simulink model "nms_sim_2D_cost"  (R2024b)
settings: Solver=ode15s  StartTime=0.0  StopTime=t_sim  MaxStep=dt_max  EnableMultiTasking=on
values from neighbouring files (symbols this model uses):
  a_BFSH = param_ctrl(35)*1    [setCtrlPar_optim_CPGreflex2001_2D.m]
  a_GAS = param_ctrl(37)*1    [setCtrlPar_optim_CPGreflex2001_2D.m]
  a_GLU = param_ctrl(31)*1    [setCtrlPar_optim_CPGreflex2001_2D.m]
  a_HAM = param_ctrl(33)*1    [setCtrlPar_optim_CPGreflex2001_2D.m]
  a_HFL = param_ctrl(32)*1    [setCtrlPar_optim_CPGreflex2001_2D.m]
  a_RF = param_ctrl(34)*1    [setCtrlPar_optim_CPGreflex2001_2D.m]
  a_SOL = param_ctrl(38)*1    [setCtrlPar_optim_CPGreflex2001_2D.m]
  a_TA = param_ctrl(39)*1    [setCtrlPar_optim_CPGreflex2001_2D.m]
  a_VAS = param_ctrl(36)*1    [setCtrlPar_optim_CPGreflex2001_2D.m]
  ai = param_ctrl(96)*2.0    [setCtrlPar_optim_CPGreflex2001_2D.m]
  b_BFSH = param_ctrl(52)*.51    [setCtrlPar_optim_CPGreflex2001_2D.m]
  b_BFSHGAS = param_ctrl(55)*.51    [setCtrlPar_optim_CPGreflex2001_2D.m]
  b_BFSHHAM = param_ctrl(54)*.51    [setCtrlPar_optim_CPGreflex2001_2D.m]
  b_BFSHVAS = param_ctrl(53)*.51    [setCtrlPar_optim_CPGreflex2001_2D.m]
  b_GAS = param_ctrl(59)*.51    [setCtrlPar_optim_CPGreflex2001_2D.m]
  b_GASBFSH = param_ctrl(60)*.51    [setCtrlPar_optim_CPGreflex2001_2D.m]
  b_GASSOL = param_ctrl(61)*.51    [setCtrlPar_optim_CPGreflex2001_2D.m]
  b_GLU = param_ctrl(40)*.51    [setCtrlPar_optim_CPGreflex2001_2D.m]
  b_GLUHAM = param_ctrl(42)*.51    [setCtrlPar_optim_CPGreflex2001_2D.m]
  b_GLUHFL = param_ctrl(41)*.51    [setCtrlPar_optim_CPGreflex2001_2D.m]
  b_HAM = param_ctrl(46)*.51    [setCtrlPar_optim_CPGreflex2001_2D.m]
  b_HAMBFSH = param_ctrl(48)*.51    [setCtrlPar_optim_CPGreflex2001_2D.m]
  b_HAMGLU = param_ctrl(47)*.51    [setCtrlPar_optim_CPGreflex2001_2D.m]
  b_HFL = param_ctrl(43)*.51    [setCtrlPar_optim_CPGreflex2001_2D.m]
  b_HFLGLU = param_ctrl(44)*.51    [setCtrlPar_optim_CPGreflex2001_2D.m]
  b_HFLRF = param_ctrl(45)*.51    [setCtrlPar_optim_CPGreflex2001_2D.m]
  b_RF = param_ctrl(49)*.51    [setCtrlPar_optim_CPGreflex2001_2D.m]
  b_RFHFL = param_ctrl(50)*.51    [setCtrlPar_optim_CPGreflex2001_2D.m]
  b_RFVAS = param_ctrl(51)*.51    [setCtrlPar_optim_CPGreflex2001_2D.m]
  b_SOL = param_ctrl(62)*.51    [setCtrlPar_optim_CPGreflex2001_2D.m]
  b_SOLGAS = param_ctrl(64)*.51    [setCtrlPar_optim_CPGreflex2001_2D.m]
  b_SOLTA = param_ctrl(63)*.51    [setCtrlPar_optim_CPGreflex2001_2D.m]
  b_TA = param_ctrl(65)*.51    [setCtrlPar_optim_CPGreflex2001_2D.m]
  b_TASOL = param_ctrl(66)*.51    [setCtrlPar_optim_CPGreflex2001_2D.m]
  b_VAS = param_ctrl(56)*.51    [setCtrlPar_optim_CPGreflex2001_2D.m]
  b_VASBFSH = param_ctrl(57)*.51    [setCtrlPar_optim_CPGreflex2001_2D.m]
  b_VASRF = param_ctrl(58)*.51    [setCtrlPar_optim_CPGreflex2001_2D.m]
  bias = param_ctrl(97)*2.5    [setCtrlPar_optim_CPGreflex2001_2D.m]
  c = 0.05    [nms_MS_2D_scaled.m]
  c_jointstop = 0.3 / (pi/180)    (= 17.1887338539)    [nms_MS_2D_scaled.m]
  D12_F = 0.16    *scaleL_JPhys    [nms_MechInit_2D_scaleSkel.m]
  D12_S = 0.2460	*sub_height    [nms_MechInit_2D_scaleSkel.m]
  D12_T = 0.2450  *sub_height    [nms_MechInit_2D_scaleSkel.m]
  D12y_F = 0.039  *sub_height    [nms_MechInit_2D_scaleSkel.m]
  D12z_HAT = 0.1    [nms_MS_2D_scaled.m]
  D13_F = 0.20    *scaleL_JPhys    [nms_MechInit_2D_scaleSkel.m]
  D1G_F = 0.14    *scaleL_JPhys    [nms_MechInit_2D_scaleSkel.m]
  D1G_HAT = 0.35  *scaleL_JPhys    [nms_MechInit_2D_scaleSkel.m]
  D1G_S = (0.3 - D12y_F/4)	*scaleL_JPhys    [nms_MechInit_2D_scaleSkel.m]
  D1G_T = (0.3 - D12y_F/4)	*scaleL_JPhys    [nms_MechInit_2D_scaleSkel.m]
  D1Gy_F = D12y_F*D1G_F/D12_F    (= 0.07)    [nms_MechInit_2D_scaleSkel.m]
  d_BFSH = param_ctrl(26)*1    [setCtrlPar_optim_CPGreflex2001_2D.m]
  d_GAS = param_ctrl(28)*1    [setCtrlPar_optim_CPGreflex2001_2D.m]
  d_GLU = param_ctrl(22)*1    [setCtrlPar_optim_CPGreflex2001_2D.m]
  d_HAM = param_ctrl(24)*1    [setCtrlPar_optim_CPGreflex2001_2D.m]
  d_HFL = param_ctrl(23)*1    [setCtrlPar_optim_CPGreflex2001_2D.m]
  d_RF = param_ctrl(25)*1    [setCtrlPar_optim_CPGreflex2001_2D.m]
  d_SOL = param_ctrl(29)*1    [setCtrlPar_optim_CPGreflex2001_2D.m]
  d_TA = param_ctrl(30)*1    [setCtrlPar_optim_CPGreflex2001_2D.m]
  d_VAS = param_ctrl(27)*1    [setCtrlPar_optim_CPGreflex2001_2D.m]
  DeltaThRef = 5e-3    (= 0.005)    [nms_MS_2D_scaled.m]
  dloptBFSH = 3.0    (= 3)    [setCtrlPar_optim_CPGreflex2001_2D.m]
  dloptGAS = 3.0    (= 3)    [setCtrlPar_optim_CPGreflex2001_2D.m]
  dloptGLU = 3.0    (= 3)    [setCtrlPar_optim_CPGreflex2001_2D.m]
  dloptHAM = 3.0    (= 3)    [setCtrlPar_optim_CPGreflex2001_2D.m]
  dloptHFL = 3.0    (= 3)    [setCtrlPar_optim_CPGreflex2001_2D.m]
  dloptRF = 3.0    (= 3)    [setCtrlPar_optim_CPGreflex2001_2D.m]
  dloptSOL = 3.0    (= 3)    [setCtrlPar_optim_CPGreflex2001_2D.m]
  dloptTA = 3.0    (= 3)    [setCtrlPar_optim_CPGreflex2001_2D.m]
  dloptVAS = 3.0    (= 3)    [setCtrlPar_optim_CPGreflex2001_2D.m]
  ec_BFSH = param_ctrl(80)*0.15    [setCtrlPar_optim_CPGreflex2001_2D.m]
  ec_GAS = param_ctrl(82)*0.15    [setCtrlPar_optim_CPGreflex2001_2D.m]
  ec_GLU = param_ctrl(76)*0.15    [setCtrlPar_optim_CPGreflex2001_2D.m]
  ec_HAM = param_ctrl(78)*0.15    [setCtrlPar_optim_CPGreflex2001_2D.m]
  ec_HFL = param_ctrl(77)*0.15    [setCtrlPar_optim_CPGreflex2001_2D.m]
  ec_RF = param_ctrl(79)*0.15    [setCtrlPar_optim_CPGreflex2001_2D.m]
  ec_TA = param_ctrl(84)*0.15    [setCtrlPar_optim_CPGreflex2001_2D.m]
  ec_VAS = param_ctrl(81)*0.15    [setCtrlPar_optim_CPGreflex2001_2D.m]
  eref = 0.04    [nms_MS_2D_scaled.m]
  eref_GAS = 0.1    [nms_MS_2D_scaled.m]
  eref_SOL = 0.1    [nms_MS_2D_scaled.m]
  es_BFSH = param_ctrl(89)*0.15    [setCtrlPar_optim_CPGreflex2001_2D.m]
  es_GAS = param_ctrl(91)*0.15    [setCtrlPar_optim_CPGreflex2001_2D.m]
  es_GLU = param_ctrl(85)*0.15    [setCtrlPar_optim_CPGreflex2001_2D.m]
  es_HAM = param_ctrl(87)*0.15    [setCtrlPar_optim_CPGreflex2001_2D.m]
  es_HFL = param_ctrl(86)*0.15    [setCtrlPar_optim_CPGreflex2001_2D.m]
  es_RF = param_ctrl(88)*0.15    [setCtrlPar_optim_CPGreflex2001_2D.m]
  es_TA = param_ctrl(93)*0.15    [setCtrlPar_optim_CPGreflex2001_2D.m]
  es_VAS = param_ctrl(90)*0.15    [setCtrlPar_optim_CPGreflex2001_2D.m]
  FmaxBFSH = 350    [nms_MS_2D_scaled.m]
  FmaxGAS = 2000    [nms_MS_2D_scaled.m]
  FmaxGLU = 4000    [nms_MS_2D_scaled.m]
  FmaxHAM = 2000    [nms_MS_2D_scaled.m]
  FmaxHFL = 2000    [nms_MS_2D_scaled.m]
  FmaxRF = 850    [nms_MS_2D_scaled.m]
  FmaxSOL = 4000    [nms_MS_2D_scaled.m]
  FmaxTA = 800    [nms_MS_2D_scaled.m]
  FmaxVAS = 5000    [nms_MS_2D_scaled.m]
  g = 9.81    [nms_MS_2D_scaled.m]
  gamma_4 = param_ctrl(11) * 1.7    [setCtrlPar_optim_CPGreflexsynergy2023_2D.m]
  h_BFSH = param_ctrl(71)*.1    [setCtrlPar_optim_CPGreflex2001_2D.m]
  h_GAS = param_ctrl(73)*.1    [setCtrlPar_optim_CPGreflex2001_2D.m]
  h_GLU = param_ctrl(67)*.1    [setCtrlPar_optim_CPGreflex2001_2D.m]
  h_HAM = param_ctrl(69)*.1    [setCtrlPar_optim_CPGreflex2001_2D.m]
  h_HFL = param_ctrl(68)*.1    [setCtrlPar_optim_CPGreflex2001_2D.m]
  h_RF = param_ctrl(70)*.1    [setCtrlPar_optim_CPGreflex2001_2D.m]
  h_SOL = param_ctrl(74)*.1    [setCtrlPar_optim_CPGreflex2001_2D.m]
  h_TA = param_ctrl(75)*.1    [setCtrlPar_optim_CPGreflex2001_2D.m]
  h_VAS = param_ctrl(72)*.1    [setCtrlPar_optim_CPGreflex2001_2D.m]
  HLCtrlPar = [theta_tgt l_clr alpha_tgt alpha_cd alpha_cv]    [setCtrlPar_optim_reflex2015_2D.m]
  In_F = 0.005    *scaleM*scaleL_JPhys^2    [nms_MechInit_2D_scaleSkel.m]
  In_HAT = 2.5    *scaleM*scaleL_JPhys^2    [nms_MechInit_2D_scaleSkel.m]
  In_S = 0.05     *scaleM*scaleL_JPhys^2    [nms_MechInit_2D_scaleSkel.m]
  In_T = 0.15     *scaleM*scaleL_JPhys^2    [nms_MechInit_2D_scaleSkel.m]
  init_exc = 0.01    [setInitPar_optim_2D.m]
  init_fm = 0.01    [setInitPar_optim_2D.m]
  init_lce = 1    [setInitPar_optim_2D.m]
  init_LCPG = param_ctrl(12) * 0.01    [setCtrlPar_optim_CPGreflexsynergy2023_2D.m]
  init_LStance = 1    [setInitPar_optim_2D.m]
  init_N1 = osc_signal1(phi_off_osc_ind)    [setCtrlPar_optim_CPGreflex2001_2D.m]
  ... (+441 more)
undefined symbols (not defined in the file or in its folder): cost_act_exponent, cost_v_tgt, flag_controller, Newton, nStep_obj, nStep_startKin, Raphson, sgn, SSW_kin, terrain_slope_angle, v_plateS1, X, Y, Z
libraries: nesl_utility x94, sm_lib x90, simulink x28, simulink_extras x12
(part 14 of 20)

== system nms_sim_2D_cost/CPG-reflex-synergy controller/Reflexes1/IN RC25 ==
  in : Inport
  Constant : Constant  Value=tau_act_diRusso
  Divide : Product  Inputs=*/
  Integrator : Integrator  InitialCondition=init_exc
  Sum : Sum  Inputs=+-|
  out : Outport  VectorParamsAs1DForOutWhenUnconnected=off
  wires:
  Constant/1 -> Divide/2
  in/1 -> Sum/1
  Integrator/1 -> out/1, Sum/2  "A"
  Divide/1 -> Integrator/1  "dA"
  Sum/1 -> Divide/1

== system nms_sim_2D_cost/CPG-reflex-synergy controller/Reflexes1/IN RC26 ==
  in : Inport
  Constant : Constant  Value=tau_act_diRusso
  Divide : Product  Inputs=*/
  Integrator : Integrator  InitialCondition=init_exc
  Sum : Sum  Inputs=+-|
  out : Outport  VectorParamsAs1DForOutWhenUnconnected=off
  wires:
  Constant/1 -> Divide/2
  in/1 -> Sum/1
  Integrator/1 -> out/1, Sum/2  "A"
  Divide/1 -> Integrator/1  "dA"
  Sum/1 -> Divide/1

== system nms_sim_2D_cost/CPG-reflex-synergy controller/Reflexes1/IN RC27 ==
  in : Inport
  Constant : Constant  Value=tau_act_diRusso
  Divide : Product  Inputs=*/
  Integrator : Integrator  InitialCondition=init_exc
  Sum : Sum  Inputs=+-|
  out : Outport  VectorParamsAs1DForOutWhenUnconnected=off
  wires:
  Constant/1 -> Divide/2
  in/1 -> Sum/1
  Integrator/1 -> out/1, Sum/2  "A"
  Divide/1 -> Integrator/1  "dA"
  Sum/1 -> Divide/1

== system nms_sim_2D_cost/CPG-reflex-synergy controller/Reflexes1/IN RC28 ==
  in : Inport
  Constant : Constant  Value=tau_act_diRusso
  Divide : Product  Inputs=*/
  Integrator : Integrator  InitialCondition=init_exc
  Sum : Sum  Inputs=+-|
  out : Outport  VectorParamsAs1DForOutWhenUnconnected=off
  wires:
  Constant/1 -> Divide/2
  in/1 -> Sum/1
  Integrator/1 -> out/1, Sum/2  "A"
  Divide/1 -> Integrator/1  "dA"
  Sum/1 -> Divide/1

== system nms_sim_2D_cost/CPG-reflex-synergy controller/Reflexes1/IN RC29 ==
  in : Inport
  Constant : Constant  Value=tau_act_diRusso
  Divide : Product  Inputs=*/
  Integrator : Integrator  InitialCondition=init_exc
  Sum : Sum  Inputs=+-|
  out : Outport  VectorParamsAs1DForOutWhenUnconnected=off
  wires:
  Constant/1 -> Divide/2
  in/1 -> Sum/1
  Integrator/1 -> out/1, Sum/2  "A"
  Divide/1 -> Integrator/1  "dA"
  Sum/1 -> Divide/1

== system nms_sim_2D_cost/CPG-reflex-synergy controller/Reflexes1/IN RC3 ==
  in : Inport
  Constant : Constant  Value=tau_act_diRusso
  Divide : Product  Inputs=*/
  Integrator : Integrator  InitialCondition=init_exc
  Sum : Sum  Inputs=+-|
  out : Outport  VectorParamsAs1DForOutWhenUnconnected=off
  wires:
  Constant/1 -> Divide/2
  in/1 -> Sum/1
  Integrator/1 -> out/1, Sum/2  "A"
  Divide/1 -> Integrator/1  "dA"
  Sum/1 -> Divide/1

== system nms_sim_2D_cost/CPG-reflex-synergy controller/Reflexes1/IN RC30 ==
  in : Inport
  Constant : Constant  Value=tau_act_diRusso
  Divide : Product  Inputs=*/
  Integrator : Integrator  InitialCondition=init_exc
  Sum : Sum  Inputs=+-|
  out : Outport  VectorParamsAs1DForOutWhenUnconnected=off
  wires:
  Constant/1 -> Divide/2
  in/1 -> Sum/1
  Integrator/1 -> out/1, Sum/2  "A"
  Divide/1 -> Integrator/1  "dA"
  Sum/1 -> Divide/1

== system nms_sim_2D_cost/CPG-reflex-synergy controller/Reflexes1/IN RC31 ==
  in : Inport
  Constant : Constant  Value=tau_act_diRusso
  Divide : Product  Inputs=*/
  Integrator : Integrator  InitialCondition=init_exc
  Sum : Sum  Inputs=+-|
  out : Outport  VectorParamsAs1DForOutWhenUnconnected=off
  wires:
  Constant/1 -> Divide/2
  in/1 -> Sum/1
  Integrator/1 -> out/1, Sum/2  "A"
  Divide/1 -> Integrator/1  "dA"
  Sum/1 -> Divide/1

== system nms_sim_2D_cost/CPG-reflex-synergy controller/Reflexes1/IN RC32 ==
  in : Inport
  Constant : Constant  Value=tau_act_diRusso
  Divide : Product  Inputs=*/
  Integrator : Integrator  InitialCondition=init_exc
  Sum : Sum  Inputs=+-|
  out : Outport  VectorParamsAs1DForOutWhenUnconnected=off
  wires:
  Constant/1 -> Divide/2
  in/1 -> Sum/1
  Integrator/1 -> out/1, Sum/2  "A"
  Divide/1 -> Integrator/1  "dA"
  Sum/1 -> Divide/1

== system nms_sim_2D_cost/CPG-reflex-synergy controller/Reflexes1/IN RC33 ==
  in : Inport
  Constant : Constant  Value=tau_act_diRusso
  Divide : Product  Inputs=*/
  Integrator : Integrator  InitialCondition=init_exc
  Sum : Sum  Inputs=+-|
  out : Outport  VectorParamsAs1DForOutWhenUnconnected=off
  wires:
  Constant/1 -> Divide/2
  in/1 -> Sum/1
  Integrator/1 -> out/1, Sum/2  "A"
  Divide/1 -> Integrator/1  "dA"
  Sum/1 -> Divide/1

== system nms_sim_2D_cost/CPG-reflex-synergy controller/Reflexes1/IN RC34 ==
  in : Inport
  Constant : Constant  Value=tau_act_diRusso
  Divide : Product  Inputs=*/
  Integrator : Integrator  InitialCondition=init_exc
  Sum : Sum  Inputs=+-|
  out : Outport  VectorParamsAs1DForOutWhenUnconnected=off
  wires:
  Constant/1 -> Divide/2
  in/1 -> Sum/1
  Integrator/1 -> out/1, Sum/2  "A"
  Divide/1 -> Integrator/1  "dA"
  Sum/1 -> Divide/1

== system nms_sim_2D_cost/CPG-reflex-synergy controller/Reflexes1/IN RC35 ==
  in : Inport
  Constant : Constant  Value=tau_act_diRusso
  Divide : Product  Inputs=*/
  Integrator : Integrator  InitialCondition=init_exc
  Sum : Sum  Inputs=+-|
  out : Outport  VectorParamsAs1DForOutWhenUnconnected=off
  wires:
  Constant/1 -> Divide/2
  in/1 -> Sum/1
  Integrator/1 -> out/1, Sum/2  "A"
  Divide/1 -> Integrator/1  "dA"
  Sum/1 -> Divide/1

== system nms_sim_2D_cost/CPG-reflex-synergy controller/Reflexes1/IN RC36 ==
  in : Inport
  Constant : Constant  Value=tau_act_diRusso
  Divide : Product  Inputs=*/
  Integrator : Integrator  InitialCondition=init_exc
  Sum : Sum  Inputs=+-|
  out : Outport  VectorParamsAs1DForOutWhenUnconnected=off
  wires:
  Constant/1 -> Divide/2
  in/1 -> Sum/1
  Integrator/1 -> out/1, Sum/2  "A"
  Divide/1 -> Integrator/1  "dA"
  Sum/1 -> Divide/1

== system nms_sim_2D_cost/CPG-reflex-synergy controller/Reflexes1/IN RC37 ==
  in : Inport
  Constant : Constant  Value=tau_act_diRusso
  Divide : Product  Inputs=*/
  Integrator : Integrator  InitialCondition=init_exc
  Sum : Sum  Inputs=+-|
  out : Outport  VectorParamsAs1DForOutWhenUnconnected=off
  wires:
  Constant/1 -> Divide/2
  in/1 -> Sum/1
  Integrator/1 -> out/1, Sum/2  "A"
  Divide/1 -> Integrator/1  "dA"
  Sum/1 -> Divide/1

== system nms_sim_2D_cost/CPG-reflex-synergy controller/Reflexes1/IN RC38 ==
  in : Inport
  Constant : Constant  Value=tau_act_diRusso
  Divide : Product  Inputs=*/
  Integrator : Integrator  InitialCondition=init_exc
  Sum : Sum  Inputs=+-|
  out : Outport  VectorParamsAs1DForOutWhenUnconnected=off
  wires:
  Constant/1 -> Divide/2
  in/1 -> Sum/1
  Integrator/1 -> out/1, Sum/2  "A"
  Divide/1 -> Integrator/1  "dA"
  Sum/1 -> Divide/1

== system nms_sim_2D_cost/CPG-reflex-synergy controller/Reflexes1/IN RC39 ==
  in : Inport
  Constant : Constant  Value=tau_act_diRusso
  Divide : Product  Inputs=*/
  Integrator : Integrator  InitialCondition=init_exc
  Sum : Sum  Inputs=+-|
  out : Outport  VectorParamsAs1DForOutWhenUnconnected=off
  wires:
  Constant/1 -> Divide/2
  in/1 -> Sum/1
  Integrator/1 -> out/1, Sum/2  "A"
  Divide/1 -> Integrator/1  "dA"
  Sum/1 -> Divide/1

== system nms_sim_2D_cost/CPG-reflex-synergy controller/Reflexes1/IN RC4 ==
  in : Inport
  Constant : Constant  Value=tau_act_diRusso
  Divide : Product  Inputs=*/
  Integrator : Integrator  InitialCondition=init_exc
  Sum : Sum  Inputs=+-|
  out : Outport  VectorParamsAs1DForOutWhenUnconnected=off
  wires:
  Constant/1 -> Divide/2
  in/1 -> Sum/1
  Integrator/1 -> out/1, Sum/2  "A"
  Divide/1 -> Integrator/1  "dA"
  Sum/1 -> Divide/1

== system nms_sim_2D_cost/CPG-reflex-synergy controller/Reflexes1/IN RC40 ==
  in : Inport
  Constant : Constant  Value=tau_act_diRusso
  Divide : Product  Inputs=*/
  Integrator : Integrator  InitialCondition=init_exc
  Sum : Sum  Inputs=+-|
  out : Outport  VectorParamsAs1DForOutWhenUnconnected=off
  wires:
  Constant/1 -> Divide/2
  in/1 -> Sum/1
  Integrator/1 -> out/1, Sum/2  "A"
  Divide/1 -> Integrator/1  "dA"
  Sum/1 -> Divide/1

== system nms_sim_2D_cost/CPG-reflex-synergy controller/Reflexes1/IN RC41 ==
  in : Inport
  Constant : Constant  Value=tau_act_diRusso
  Divide : Product  Inputs=*/
  Integrator : Integrator  InitialCondition=init_exc
  Sum : Sum  Inputs=+-|
  out : Outport  VectorParamsAs1DForOutWhenUnconnected=off
  wires:
  Constant/1 -> Divide/2
  in/1 -> Sum/1
  Integrator/1 -> out/1, Sum/2  "A"
  Divide/1 -> Integrator/1  "dA"
  Sum/1 -> Divide/1

== system nms_sim_2D_cost/CPG-reflex-synergy controller/Reflexes1/IN RC42 ==
  in : Inport
  Constant : Constant  Value=tau_act_diRusso
  Divide : Product  Inputs=*/
  Integrator : Integrator  InitialCondition=init_exc
  Sum : Sum  Inputs=+-|
  out : Outport  VectorParamsAs1DForOutWhenUnconnected=off
  wires:
  Constant/1 -> Divide/2
  in/1 -> Sum/1
  Integrator/1 -> out/1, Sum/2  "A"
  Divide/1 -> Integrator/1  "dA"
  Sum/1 -> Divide/1

== system nms_sim_2D_cost/CPG-reflex-synergy controller/Reflexes1/IN RC43 ==
  in : Inport
  Constant : Constant  Value=tau_act_diRusso
  Divide : Product  Inputs=*/
  Integrator : Integrator  InitialCondition=init_exc
  Sum : Sum  Inputs=+-|
  out : Outport  VectorParamsAs1DForOutWhenUnconnected=off
  wires:
  Constant/1 -> Divide/2
  in/1 -> Sum/1
  Integrator/1 -> out/1, Sum/2  "A"
  Divide/1 -> Integrator/1  "dA"
  Sum/1 -> Divide/1

== system nms_sim_2D_cost/CPG-reflex-synergy controller/Reflexes1/IN RC44 ==
  in : Inport
  Constant : Constant  Value=tau_act_diRusso
  Divide : Product  Inputs=*/
  Integrator : Integrator  InitialCondition=init_exc
  Sum : Sum  Inputs=+-|
  out : Outport  VectorParamsAs1DForOutWhenUnconnected=off
  wires:
  Constant/1 -> Divide/2
  in/1 -> Sum/1
  Integrator/1 -> out/1, Sum/2  "A"
  Divide/1 -> Integrator/1  "dA"
  Sum/1 -> Divide/1

== system nms_sim_2D_cost/CPG-reflex-synergy controller/Reflexes1/IN RC45 ==
  in : Inport
  Constant : Constant  Value=tau_act_diRusso
  Divide : Product  Inputs=*/
  Integrator : Integrator  InitialCondition=init_exc
  Sum : Sum  Inputs=+-|
  out : Outport  VectorParamsAs1DForOutWhenUnconnected=off
  wires:
  Constant/1 -> Divide/2
  in/1 -> Sum/1
  Integrator/1 -> out/1, Sum/2  "A"
  Divide/1 -> Integrator/1  "dA"
  Sum/1 -> Divide/1

== system nms_sim_2D_cost/CPG-reflex-synergy controller/Reflexes1/IN RC46 ==
  in : Inport
  Constant : Constant  Value=tau_act_diRusso
  Divide : Product  Inputs=*/
  Integrator : Integrator  InitialCondition=init_exc
  Sum : Sum  Inputs=+-|
  out : Outport  VectorParamsAs1DForOutWhenUnconnected=off
  wires:
  Constant/1 -> Divide/2
  in/1 -> Sum/1
  Integrator/1 -> out/1, Sum/2  "A"
  Divide/1 -> Integrator/1  "dA"
  Sum/1 -> Divide/1

== system nms_sim_2D_cost/CPG-reflex-synergy controller/Reflexes1/IN RC47 ==
  in : Inport
  Constant : Constant  Value=tau_act_diRusso
  Divide : Product  Inputs=*/
  Integrator : Integrator  InitialCondition=init_exc
  Sum : Sum  Inputs=+-|
  out : Outport  VectorParamsAs1DForOutWhenUnconnected=off
  wires:
  Constant/1 -> Divide/2
  in/1 -> Sum/1
  Integrator/1 -> out/1, Sum/2  "A"
  Divide/1 -> Integrator/1  "dA"
  Sum/1 -> Divide/1

== system nms_sim_2D_cost/CPG-reflex-synergy controller/Reflexes1/IN RC48 ==
  in : Inport
  Constant : Constant  Value=tau_act_diRusso
  Divide : Product  Inputs=*/
  Integrator : Integrator  InitialCondition=init_exc
  Sum : Sum  Inputs=+-|
  out : Outport  VectorParamsAs1DForOutWhenUnconnected=off
  wires:
  Constant/1 -> Divide/2
  in/1 -> Sum/1
  Integrator/1 -> out/1, Sum/2  "A"
  Divide/1 -> Integrator/1  "dA"
  Sum/1 -> Divide/1

== system nms_sim_2D_cost/CPG-reflex-synergy controller/Reflexes1/IN RC49 ==
  in : Inport
  Constant : Constant  Value=tau_act_diRusso
  Divide : Product  Inputs=*/
  Integrator : Integrator  InitialCondition=init_exc
  Sum : Sum  Inputs=+-|
  out : Outport  VectorParamsAs1DForOutWhenUnconnected=off
  wires:
  Constant/1 -> Divide/2
  in/1 -> Sum/1
  Integrator/1 -> out/1, Sum/2  "A"
  Divide/1 -> Integrator/1  "dA"
  Sum/1 -> Divide/1

== system nms_sim_2D_cost/CPG-reflex-synergy controller/Reflexes1/IN RC5 ==
  in : Inport
  Constant : Constant  Value=tau_act_diRusso
  Divide : Product  Inputs=*/
  Integrator : Integrator  InitialCondition=init_exc
  Sum : Sum  Inputs=+-|
  out : Outport  VectorParamsAs1DForOutWhenUnconnected=off
  wires:
  Constant/1 -> Divide/2
  in/1 -> Sum/1
  Integrator/1 -> out/1, Sum/2  "A"
  Divide/1 -> Integrator/1  "dA"
  Sum/1 -> Divide/1

== system nms_sim_2D_cost/CPG-reflex-synergy controller/Reflexes1/IN RC50 ==
  in : Inport
  Constant : Constant  Value=tau_act_diRusso
  Divide : Product  Inputs=*/
  Integrator : Integrator  InitialCondition=init_exc
  Sum : Sum  Inputs=+-|
  out : Outport  VectorParamsAs1DForOutWhenUnconnected=off
  wires:
  Constant/1 -> Divide/2
  in/1 -> Sum/1
  Integrator/1 -> out/1, Sum/2  "A"
  Divide/1 -> Integrator/1  "dA"
  Sum/1 -> Divide/1

== system nms_sim_2D_cost/CPG-reflex-synergy controller/Reflexes1/IN RC51 ==
  in : Inport
  Constant : Constant  Value=tau_act_diRusso
  Divide : Product  Inputs=*/
  Integrator : Integrator  InitialCondition=init_exc
  Sum : Sum  Inputs=+-|
  out : Outport  VectorParamsAs1DForOutWhenUnconnected=off
  wires:
  Constant/1 -> Divide/2
  in/1 -> Sum/1
  Integrator/1 -> out/1, Sum/2  "A"
  Divide/1 -> Integrator/1  "dA"
  Sum/1 -> Divide/1

== system nms_sim_2D_cost/CPG-reflex-synergy controller/Reflexes1/IN RC6 ==
  in : Inport
  Constant : Constant  Value=tau_act_diRusso
  Divide : Product  Inputs=*/
  Integrator : Integrator  InitialCondition=init_exc
  Sum : Sum  Inputs=+-|
  out : Outport  VectorParamsAs1DForOutWhenUnconnected=off
  wires:
  Constant/1 -> Divide/2
  in/1 -> Sum/1
  Integrator/1 -> out/1, Sum/2  "A"
  Divide/1 -> Integrator/1  "dA"
  Sum/1 -> Divide/1

== system nms_sim_2D_cost/CPG-reflex-synergy controller/Reflexes1/IN RC7 ==
  in : Inport
  Constant : Constant  Value=tau_act_diRusso
  Divide : Product  Inputs=*/
  Integrator : Integrator  InitialCondition=init_exc
  Sum : Sum  Inputs=+-|
  out : Outport  VectorParamsAs1DForOutWhenUnconnected=off
  wires:
  Constant/1 -> Divide/2
  in/1 -> Sum/1
  Integrator/1 -> out/1, Sum/2  "A"
  Divide/1 -> Integrator/1  "dA"
  Sum/1 -> Divide/1

== system nms_sim_2D_cost/CPG-reflex-synergy controller/Reflexes1/IN RC8 ==
  in : Inport
  Constant : Constant  Value=tau_act_diRusso
  Divide : Product  Inputs=*/
  Integrator : Integrator  InitialCondition=init_exc
  Sum : Sum  Inputs=+-|
  out : Outport  VectorParamsAs1DForOutWhenUnconnected=off
  wires:
  Sum/1 -> Divide/1
  Divide/1 -> Integrator/1  "dA"
  Integrator/1 -> Sum/2, out/1  "A"
  in/1 -> Sum/1
  Constant/1 -> Divide/2

== system nms_sim_2D_cost/CPG-reflex-synergy controller/Reflexes1/IN RC9 ==
  in : Inport
  Constant : Constant  Value=tau_act_diRusso
  Divide : Product  Inputs=*/
  Integrator : Integrator  InitialCondition=init_exc
  Sum : Sum  Inputs=+-|
  out : Outport  VectorParamsAs1DForOutWhenUnconnected=off
  wires:
  Constant/1 -> Divide/2
  in/1 -> Sum/1
  Integrator/1 -> out/1, Sum/2  "A"
  Divide/1 -> Integrator/1  "dA"
  Sum/1 -> Divide/1

== system nms_sim_2D_cost/CPG-reflex-synergy controller/Reflexes1/SN ==
  In1 : Inport
  Gain : Gain  Gain=65/200
  Sqrt : Sqrt
  Out1 : Outport
  wires:
  In1/1 -> Sqrt/1
  Sqrt/1 -> Gain/1
  Gain/1 -> Out1/1

== system nms_sim_2D_cost/CPG-reflex-synergy controller/Reflexes1/SN1 ==
  In1 : Inport
  Gain : Gain  Gain=65/200
  Sqrt : Sqrt
  Out1 : Outport
  wires:
  Gain/1 -> Out1/1
  Sqrt/1 -> Gain/1
  In1/1 -> Sqrt/1

== system nms_sim_2D_cost/CPG-reflex-synergy controller/Reflexes1/SN2 ==
  In1 : Inport
  Gain : Gain  Gain=65/200
  Sqrt : Sqrt
  Out1 : Outport
  wires:
  In1/1 -> Sqrt/1
  Sqrt/1 -> Gain/1
  Gain/1 -> Out1/1

== system nms_sim_2D_cost/CPG-reflex-synergy controller/Reflexes1/SN3 ==
  In1 : Inport
  Gain : Gain  Gain=65/200
  Sqrt : Sqrt
  Out1 : Outport
  wires:
  Gain/1 -> Out1/1
  Sqrt/1 -> Gain/1
  In1/1 -> Sqrt/1

== system nms_sim_2D_cost/CPG-reflex-synergy controller/Reflexes1/SN4 ==
  In1 : Inport
  Gain : Gain  Gain=65/200
  Sqrt : Sqrt
  Out1 : Outport
  wires:
  In1/1 -> Sqrt/1
  Sqrt/1 -> Gain/1
  Gain/1 -> Out1/1

== system nms_sim_2D_cost/CPG-reflex-synergy controller/Reflexes1/SN5 ==
  In1 : Inport
  Gain : Gain  Gain=65/200
  Sqrt : Sqrt
  Out1 : Outport
  wires:
  Gain/1 -> Out1/1
  Sqrt/1 -> Gain/1
  In1/1 -> Sqrt/1

== system nms_sim_2D_cost/CPG-reflex-synergy controller/Reflexes1/SN6 ==
  In1 : Inport
  Gain : Gain  Gain=65/200
  Sqrt : Sqrt
  Out1 : Outport
  wires:
  In1/1 -> Sqrt/1
  Sqrt/1 -> Gain/1
  Gain/1 -> Out1/1

== system nms_sim_2D_cost/CPG-reflex-synergy controller/Reflexes1/SN7 ==
  In1 : Inport
  Gain : Gain  Gain=65/200
  Sqrt : Sqrt
  Out1 : Outport
  wires:
  Gain/1 -> Out1/1
  Sqrt/1 -> Gain/1
  In1/1 -> Sqrt/1

== system nms_sim_2D_cost/CPG-reflex-synergy controller/Reflexes1/SN8 ==
  In1 : Inport
  Gain : Gain  Gain=65/200
  Sqrt : Sqrt
  Out1 : Outport
  wires:
  In1/1 -> Sqrt/1
  Sqrt/1 -> Gain/1
  Gain/1 -> Out1/1

== system nms_sim_2D_cost/CPG-reflex-synergy controller/Reflexes2/IN RC1 ==
  in : Inport
  Constant : Constant  Value=tau_act_diRusso
  Divide : Product  Inputs=*/
  Integrator : Integrator  InitialCondition=init_exc
  Sum : Sum  Inputs=+-|
  out : Outport  VectorParamsAs1DForOutWhenUnconnected=off
  wires:
  Constant/1 -> Divide/2
  in/1 -> Sum/1
  Integrator/1 -> out/1, Sum/2  "A"
  Divide/1 -> Integrator/1  "dA"
  Sum/1 -> Divide/1

== system nms_sim_2D_cost/CPG-reflex-synergy controller/Reflexes2/IN RC10 ==
  in : Inport
  Constant : Constant  Value=tau_act_diRusso
  Divide : Product  Inputs=*/
  Integrator : Integrator  InitialCondition=init_exc
  Sum : Sum  Inputs=+-|
  out : Outport  VectorParamsAs1DForOutWhenUnconnected=off
  wires:
  Constant/1 -> Divide/2
  in/1 -> Sum/1
  Integrator/1 -> out/1, Sum/2  "A"
  Divide/1 -> Integrator/1  "dA"
  Sum/1 -> Divide/1

== system nms_sim_2D_cost/CPG-reflex-synergy controller/Reflexes2/IN RC11 ==
  in : Inport
  Constant : Constant  Value=tau_act_diRusso
  Divide : Product  Inputs=*/
  Integrator : Integrator  InitialCondition=init_exc
  Sum : Sum  Inputs=+-|
  out : Outport  VectorParamsAs1DForOutWhenUnconnected=off
  wires:
  Constant/1 -> Divide/2
  in/1 -> Sum/1
  Integrator/1 -> out/1, Sum/2  "A"
  Divide/1 -> Integrator/1  "dA"
  Sum/1 -> Divide/1

== system nms_sim_2D_cost/CPG-reflex-synergy controller/Reflexes2/IN RC12 ==
  in : Inport
  Constant : Constant  Value=tau_act_diRusso
  Divide : Product  Inputs=*/
  Integrator : Integrator  InitialCondition=init_exc
  Sum : Sum  Inputs=+-|
  out : Outport  VectorParamsAs1DForOutWhenUnconnected=off
  wires:
  Constant/1 -> Divide/2
  in/1 -> Sum/1
  Integrator/1 -> out/1, Sum/2  "A"
  Divide/1 -> Integrator/1  "dA"
  Sum/1 -> Divide/1

== system nms_sim_2D_cost/CPG-reflex-synergy controller/Reflexes2/IN RC13 ==
  in : Inport
  Constant : Constant  Value=tau_act_diRusso
  Divide : Product  Inputs=*/
  Integrator : Integrator  InitialCondition=init_exc
  Sum : Sum  Inputs=+-|
  out : Outport  VectorParamsAs1DForOutWhenUnconnected=off
  wires:
  Constant/1 -> Divide/2
  in/1 -> Sum/1
  Integrator/1 -> out/1, Sum/2  "A"
  Divide/1 -> Integrator/1  "dA"
  Sum/1 -> Divide/1

== system nms_sim_2D_cost/CPG-reflex-synergy controller/Reflexes2/IN RC14 ==
  in : Inport
  Constant : Constant  Value=tau_act_diRusso
  Divide : Product  Inputs=*/
  Integrator : Integrator  InitialCondition=init_exc
  Sum : Sum  Inputs=+-|
  out : Outport  VectorParamsAs1DForOutWhenUnconnected=off
  wires:
  Constant/1 -> Divide/2
  in/1 -> Sum/1
  Integrator/1 -> out/1, Sum/2  "A"
  Divide/1 -> Integrator/1  "dA"
  Sum/1 -> Divide/1

== system nms_sim_2D_cost/CPG-reflex-synergy controller/Reflexes2/IN RC15 ==
  in : Inport
  Constant : Constant  Value=tau_act_diRusso
  Divide : Product  Inputs=*/
  Integrator : Integrator  InitialCondition=init_exc
  Sum : Sum  Inputs=+-|
  out : Outport  VectorParamsAs1DForOutWhenUnconnected=off
  wires:
  Constant/1 -> Divide/2
  in/1 -> Sum/1
  Integrator/1 -> out/1, Sum/2  "A"
  Divide/1 -> Integrator/1  "dA"
  Sum/1 -> Divide/1

== system nms_sim_2D_cost/CPG-reflex-synergy controller/Reflexes2/IN RC16 ==
  in : Inport
  Constant : Constant  Value=tau_act_diRusso
  Divide : Product  Inputs=*/
  Integrator : Integrator  InitialCondition=init_exc
  Sum : Sum  Inputs=+-|
  out : Outport  VectorParamsAs1DForOutWhenUnconnected=off
  wires:
  Constant/1 -> Divide/2
  in/1 -> Sum/1
  Integrator/1 -> out/1, Sum/2  "A"
  Divide/1 -> Integrator/1  "dA"
  Sum/1 -> Divide/1

== system nms_sim_2D_cost/CPG-reflex-synergy controller/Reflexes2/IN RC17 ==
  in : Inport
  Constant : Constant  Value=tau_act_diRusso
  Divide : Product  Inputs=*/
  Integrator : Integrator  InitialCondition=init_exc
  Sum : Sum  Inputs=+-|
  out : Outport  VectorParamsAs1DForOutWhenUnconnected=off
  wires:
  Constant/1 -> Divide/2
  in/1 -> Sum/1
  Integrator/1 -> out/1, Sum/2  "A"
  Divide/1 -> Integrator/1  "dA"
  Sum/1 -> Divide/1

== system nms_sim_2D_cost/CPG-reflex-synergy controller/Reflexes2/IN RC18 ==
  in : Inport
  Constant : Constant  Value=tau_act_diRusso
  Divide : Product  Inputs=*/
  Integrator : Integrator  InitialCondition=init_exc
  Sum : Sum  Inputs=+-|
  out : Outport  VectorParamsAs1DForOutWhenUnconnected=off
  wires:
  Constant/1 -> Divide/2
  in/1 -> Sum/1
  Integrator/1 -> out/1, Sum/2  "A"
  Divide/1 -> Integrator/1  "dA"
  Sum/1 -> Divide/1

== system nms_sim_2D_cost/CPG-reflex-synergy controller/Reflexes2/IN RC19 ==
  in : Inport
  Constant : Constant  Value=tau_act_diRusso
  Divide : Product  Inputs=*/
  Integrator : Integrator  InitialCondition=init_exc
  Sum : Sum  Inputs=+-|
  out : Outport  VectorParamsAs1DForOutWhenUnconnected=off
  wires:
  Constant/1 -> Divide/2
  in/1 -> Sum/1
  Integrator/1 -> out/1, Sum/2  "A"
  Divide/1 -> Integrator/1  "dA"
  Sum/1 -> Divide/1

== system nms_sim_2D_cost/CPG-reflex-synergy controller/Reflexes2/IN RC2 ==
  in : Inport
  Constant : Constant  Value=tau_act_diRusso
  Divide : Product  Inputs=*/
  Integrator : Integrator  InitialCondition=init_exc
  Sum : Sum  Inputs=+-|
  out : Outport  VectorParamsAs1DForOutWhenUnconnected=off
  wires:
  Constant/1 -> Divide/2
  in/1 -> Sum/1
  Integrator/1 -> out/1, Sum/2  "A"
  Divide/1 -> Integrator/1  "dA"
  Sum/1 -> Divide/1

== system nms_sim_2D_cost/CPG-reflex-synergy controller/Reflexes2/IN RC20 ==
  in : Inport
  Constant : Constant  Value=tau_act_diRusso
  Divide : Product  Inputs=*/
  Integrator : Integrator  InitialCondition=init_exc
  Sum : Sum  Inputs=+-|
  out : Outport  VectorParamsAs1DForOutWhenUnconnected=off
  wires:
  Constant/1 -> Divide/2
  in/1 -> Sum/1
  Integrator/1 -> out/1, Sum/2  "A"
  Divide/1 -> Integrator/1  "dA"
  Sum/1 -> Divide/1

== system nms_sim_2D_cost/CPG-reflex-synergy controller/Reflexes2/IN RC21 ==
  in : Inport
  Constant : Constant  Value=tau_act_diRusso
  Divide : Product  Inputs=*/
  Integrator : Integrator  InitialCondition=init_exc
  Sum : Sum  Inputs=+-|
  out : Outport  VectorParamsAs1DForOutWhenUnconnected=off
  wires:
  Constant/1 -> Divide/2
  in/1 -> Sum/1
  Integrator/1 -> out/1, Sum/2  "A"
  Divide/1 -> Integrator/1  "dA"
  Sum/1 -> Divide/1

== system nms_sim_2D_cost/CPG-reflex-synergy controller/Reflexes2/IN RC22 ==
  in : Inport
  Constant : Constant  Value=tau_act_diRusso
  Divide : Product  Inputs=*/
  Integrator : Integrator  InitialCondition=init_exc
  Sum : Sum  Inputs=+-|
  out : Outport  VectorParamsAs1DForOutWhenUnconnected=off
  wires:
  Constant/1 -> Divide/2
  in/1 -> Sum/1
  Integrator/1 -> out/1, Sum/2  "A"
  Divide/1 -> Integrator/1  "dA"
  Sum/1 -> Divide/1

== system nms_sim_2D_cost/CPG-reflex-synergy controller/Reflexes2/IN RC23 ==
  in : Inport
  Constant : Constant  Value=tau_act_diRusso
  Divide : Product  Inputs=*/
  Integrator : Integrator  InitialCondition=init_exc
  Sum : Sum  Inputs=+-|
  out : Outport  VectorParamsAs1DForOutWhenUnconnected=off
  wires:
  Constant/1 -> Divide/2
  in/1 -> Sum/1
  Integrator/1 -> out/1, Sum/2  "A"
  Divide/1 -> Integrator/1  "dA"
  Sum/1 -> Divide/1

== system nms_sim_2D_cost/CPG-reflex-synergy controller/Reflexes2/IN RC24 ==
  in : Inport
  Constant : Constant  Value=tau_act_diRusso
  Divide : Product  Inputs=*/
  Integrator : Integrator  InitialCondition=init_exc
  Sum : Sum  Inputs=+-|
  out : Outport  VectorParamsAs1DForOutWhenUnconnected=off
  wires:
  Constant/1 -> Divide/2
  in/1 -> Sum/1
  Integrator/1 -> out/1, Sum/2  "A"
  Divide/1 -> Integrator/1  "dA"
  Sum/1 -> Divide/1

== system nms_sim_2D_cost/CPG-reflex-synergy controller/Reflexes2/IN RC25 ==
  in : Inport
  Constant : Constant  Value=tau_act_diRusso
  Divide : Product  Inputs=*/
  Integrator : Integrator  InitialCondition=init_exc
  Sum : Sum  Inputs=+-|
  out : Outport  VectorParamsAs1DForOutWhenUnconnected=off
  wires:
  Constant/1 -> Divide/2
  in/1 -> Sum/1
  Integrator/1 -> out/1, Sum/2  "A"
  Divide/1 -> Integrator/1  "dA"
  Sum/1 -> Divide/1

== system nms_sim_2D_cost/CPG-reflex-synergy controller/Reflexes2/IN RC26 ==
  in : Inport
  Constant : Constant  Value=tau_act_diRusso
  Divide : Product  Inputs=*/
  Integrator : Integrator  InitialCondition=init_exc
  Sum : Sum  Inputs=+-|
  out : Outport  VectorParamsAs1DForOutWhenUnconnected=off
  wires:
  Constant/1 -> Divide/2
  in/1 -> Sum/1
  Integrator/1 -> out/1, Sum/2  "A"
  Divide/1 -> Integrator/1  "dA"
  Sum/1 -> Divide/1

== system nms_sim_2D_cost/CPG-reflex-synergy controller/Reflexes2/IN RC27 ==
  in : Inport
  Constant : Constant  Value=tau_act_diRusso
  Divide : Product  Inputs=*/
  Integrator : Integrator  InitialCondition=init_exc
  Sum : Sum  Inputs=+-|
  out : Outport  VectorParamsAs1DForOutWhenUnconnected=off
  wires:
  Constant/1 -> Divide/2
  in/1 -> Sum/1
  Integrator/1 -> out/1, Sum/2  "A"
  Divide/1 -> Integrator/1  "dA"
  Sum/1 -> Divide/1

== system nms_sim_2D_cost/CPG-reflex-synergy controller/Reflexes2/IN RC28 ==
  in : Inport
  Constant : Constant  Value=tau_act_diRusso
  Divide : Product  Inputs=*/
  Integrator : Integrator  InitialCondition=init_exc
  Sum : Sum  Inputs=+-|
  out : Outport  VectorParamsAs1DForOutWhenUnconnected=off
  wires:
  Constant/1 -> Divide/2
  in/1 -> Sum/1
  Integrator/1 -> out/1, Sum/2  "A"
  Divide/1 -> Integrator/1  "dA"
  Sum/1 -> Divide/1

== system nms_sim_2D_cost/CPG-reflex-synergy controller/Reflexes2/IN RC29 ==
  in : Inport
  Constant : Constant  Value=tau_act_diRusso
  Divide : Product  Inputs=*/
  Integrator : Integrator  InitialCondition=init_exc
  Sum : Sum  Inputs=+-|
  out : Outport  VectorParamsAs1DForOutWhenUnconnected=off
  wires:
  Constant/1 -> Divide/2
  in/1 -> Sum/1
  Integrator/1 -> out/1, Sum/2  "A"
  Divide/1 -> Integrator/1  "dA"
  Sum/1 -> Divide/1

== system nms_sim_2D_cost/CPG-reflex-synergy controller/Reflexes2/IN RC3 ==
  in : Inport
  Constant : Constant  Value=tau_act_diRusso
  Divide : Product  Inputs=*/
  Integrator : Integrator  InitialCondition=init_exc
  Sum : Sum  Inputs=+-|
  out : Outport  VectorParamsAs1DForOutWhenUnconnected=off
  wires:
  Constant/1 -> Divide/2
  in/1 -> Sum/1
  Integrator/1 -> out/1, Sum/2  "A"
  Divide/1 -> Integrator/1  "dA"
  Sum/1 -> Divide/1

== system nms_sim_2D_cost/CPG-reflex-synergy controller/Reflexes2/IN RC30 ==
  in : Inport
  Constant : Constant  Value=tau_act_diRusso
  Divide : Product  Inputs=*/
  Integrator : Integrator  InitialCondition=init_exc
  Sum : Sum  Inputs=+-|
  out : Outport  VectorParamsAs1DForOutWhenUnconnected=off
  wires:
  Constant/1 -> Divide/2
  in/1 -> Sum/1
  Integrator/1 -> out/1, Sum/2  "A"
  Divide/1 -> Integrator/1  "dA"
  Sum/1 -> Divide/1

== system nms_sim_2D_cost/CPG-reflex-synergy controller/Reflexes2/IN RC31 ==
  in : Inport
  Constant : Constant  Value=tau_act_diRusso
  Divide : Product  Inputs=*/
  Integrator : Integrator  InitialCondition=init_exc
  Sum : Sum  Inputs=+-|
  out : Outport  VectorParamsAs1DForOutWhenUnconnected=off
  wires:
  Constant/1 -> Divide/2
  in/1 -> Sum/1
  Integrator/1 -> out/1, Sum/2  "A"
  Divide/1 -> Integrator/1  "dA"
  Sum/1 -> Divide/1

== system nms_sim_2D_cost/CPG-reflex-synergy controller/Reflexes2/IN RC32 ==
  in : Inport
  Constant : Constant  Value=tau_act_diRusso
  Divide : Product  Inputs=*/
  Integrator : Integrator  InitialCondition=init_exc
  Sum : Sum  Inputs=+-|
  out : Outport  VectorParamsAs1DForOutWhenUnconnected=off
  wires:
  Constant/1 -> Divide/2
  in/1 -> Sum/1
  Integrator/1 -> out/1, Sum/2  "A"
  Divide/1 -> Integrator/1  "dA"
  Sum/1 -> Divide/1

== system nms_sim_2D_cost/CPG-reflex-synergy controller/Reflexes2/IN RC33 ==
  in : Inport
  Constant : Constant  Value=tau_act_diRusso
  Divide : Product  Inputs=*/
  Integrator : Integrator  InitialCondition=init_exc
  Sum : Sum  Inputs=+-|
  out : Outport  VectorParamsAs1DForOutWhenUnconnected=off
  wires:
  Constant/1 -> Divide/2
  in/1 -> Sum/1
  Integrator/1 -> out/1, Sum/2  "A"
  Divide/1 -> Integrator/1  "dA"
  Sum/1 -> Divide/1

== system nms_sim_2D_cost/CPG-reflex-synergy controller/Reflexes2/IN RC34 ==
  in : Inport
  Constant : Constant  Value=tau_act_diRusso
  Divide : Product  Inputs=*/
  Integrator : Integrator  InitialCondition=init_exc
  Sum : Sum  Inputs=+-|
  out : Outport  VectorParamsAs1DForOutWhenUnconnected=off
  wires:
  Constant/1 -> Divide/2
  in/1 -> Sum/1
  Integrator/1 -> out/1, Sum/2  "A"
  Divide/1 -> Integrator/1  "dA"
  Sum/1 -> Divide/1

== system nms_sim_2D_cost/CPG-reflex-synergy controller/Reflexes2/IN RC35 ==
  in : Inport
  Constant : Constant  Value=tau_act_diRusso
  Divide : Product  Inputs=*/
  Integrator : Integrator  InitialCondition=init_exc
  Sum : Sum  Inputs=+-|
  out : Outport  VectorParamsAs1DForOutWhenUnconnected=off
  wires:
  Constant/1 -> Divide/2
  in/1 -> Sum/1
  Integrator/1 -> out/1, Sum/2  "A"
  Divide/1 -> Integrator/1  "dA"
  Sum/1 -> Divide/1

== system nms_sim_2D_cost/CPG-reflex-synergy controller/Reflexes2/IN RC36 ==
  in : Inport
  Constant : Constant  Value=tau_act_diRusso
  Divide : Product  Inputs=*/
  Integrator : Integrator  InitialCondition=init_exc
  Sum : Sum  Inputs=+-|
  out : Outport  VectorParamsAs1DForOutWhenUnconnected=off
  wires:
  Constant/1 -> Divide/2
  in/1 -> Sum/1
  Integrator/1 -> out/1, Sum/2  "A"
  Divide/1 -> Integrator/1  "dA"
  Sum/1 -> Divide/1

== system nms_sim_2D_cost/CPG-reflex-synergy controller/Reflexes2/IN RC37 ==
  in : Inport
  Constant : Constant  Value=tau_act_diRusso
  Divide : Product  Inputs=*/
  Integrator : Integrator  InitialCondition=init_exc
  Sum : Sum  Inputs=+-|
  out : Outport  VectorParamsAs1DForOutWhenUnconnected=off
  wires:
  Constant/1 -> Divide/2
  in/1 -> Sum/1
  Integrator/1 -> out/1, Sum/2  "A"
  Divide/1 -> Integrator/1  "dA"
  Sum/1 -> Divide/1

== system nms_sim_2D_cost/CPG-reflex-synergy controller/Reflexes2/IN RC38 ==
  in : Inport
  Constant : Constant  Value=tau_act_diRusso
  Divide : Product  Inputs=*/
  Integrator : Integrator  InitialCondition=init_exc
  Sum : Sum  Inputs=+-|
  out : Outport  VectorParamsAs1DForOutWhenUnconnected=off
  wires:
  Constant/1 -> Divide/2
  in/1 -> Sum/1
  Integrator/1 -> out/1, Sum/2  "A"
  Divide/1 -> Integrator/1  "dA"
  Sum/1 -> Divide/1

== system nms_sim_2D_cost/CPG-reflex-synergy controller/Reflexes2/IN RC39 ==
  in : Inport
  Constant : Constant  Value=tau_act_diRusso
  Divide : Product  Inputs=*/
  Integrator : Integrator  InitialCondition=init_exc
  Sum : Sum  Inputs=+-|
  out : Outport  VectorParamsAs1DForOutWhenUnconnected=off
  wires:
  Constant/1 -> Divide/2
  in/1 -> Sum/1
  Integrator/1 -> out/1, Sum/2  "A"
  Divide/1 -> Integrator/1  "dA"
  Sum/1 -> Divide/1

== system nms_sim_2D_cost/CPG-reflex-synergy controller/Reflexes2/IN RC4 ==
  in : Inport
  Constant : Constant  Value=tau_act_diRusso
  Divide : Product  Inputs=*/
  Integrator : Integrator  InitialCondition=init_exc
  Sum : Sum  Inputs=+-|
  out : Outport  VectorParamsAs1DForOutWhenUnconnected=off
  wires:
  Constant/1 -> Divide/2
  in/1 -> Sum/1
  Integrator/1 -> out/1, Sum/2  "A"
  Divide/1 -> Integrator/1  "dA"
  Sum/1 -> Divide/1

== system nms_sim_2D_cost/CPG-reflex-synergy controller/Reflexes2/IN RC40 ==
  in : Inport
  Constant : Constant  Value=tau_act_diRusso
  Divide : Product  Inputs=*/
  Integrator : Integrator  InitialCondition=init_exc
  Sum : Sum  Inputs=+-|
  out : Outport  VectorParamsAs1DForOutWhenUnconnected=off
  wires:
  Constant/1 -> Divide/2
  in/1 -> Sum/1
  Integrator/1 -> out/1, Sum/2  "A"
  Divide/1 -> Integrator/1  "dA"
  Sum/1 -> Divide/1

== system nms_sim_2D_cost/CPG-reflex-synergy controller/Reflexes2/IN RC41 ==
  in : Inport
  Constant : Constant  Value=tau_act_diRusso
  Divide : Product  Inputs=*/
  Integrator : Integrator  InitialCondition=init_exc
  Sum : Sum  Inputs=+-|
  out : Outport  VectorParamsAs1DForOutWhenUnconnected=off
  wires:
  Constant/1 -> Divide/2
  in/1 -> Sum/1
  Integrator/1 -> out/1, Sum/2  "A"
  Divide/1 -> Integrator/1  "dA"
  Sum/1 -> Divide/1

== system nms_sim_2D_cost/CPG-reflex-synergy controller/Reflexes2/IN RC42 ==
  in : Inport
  Constant : Constant  Value=tau_act_diRusso
  Divide : Product  Inputs=*/
  Integrator : Integrator  InitialCondition=init_exc
  Sum : Sum  Inputs=+-|
  out : Outport  VectorParamsAs1DForOutWhenUnconnected=off
  wires:
  Constant/1 -> Divide/2
  in/1 -> Sum/1
  Integrator/1 -> out/1, Sum/2  "A"
  Divide/1 -> Integrator/1  "dA"
  Sum/1 -> Divide/1

== system nms_sim_2D_cost/CPG-reflex-synergy controller/Reflexes2/IN RC43 ==
  in : Inport
  Constant : Constant  Value=tau_act_diRusso
  Divide : Product  Inputs=*/
  Integrator : Integrator  InitialCondition=init_exc
  Sum : Sum  Inputs=+-|
  out : Outport  VectorParamsAs1DForOutWhenUnconnected=off
  wires:
  Constant/1 -> Divide/2
  in/1 -> Sum/1
  Integrator/1 -> out/1, Sum/2  "A"
  Divide/1 -> Integrator/1  "dA"
  Sum/1 -> Divide/1

== system nms_sim_2D_cost/CPG-reflex-synergy controller/Reflexes2/IN RC44 ==
  in : Inport
  Constant : Constant  Value=tau_act_diRusso
  Divide : Product  Inputs=*/
  Integrator : Integrator  InitialCondition=init_exc
  Sum : Sum  Inputs=+-|
  out : Outport  VectorParamsAs1DForOutWhenUnconnected=off
  wires:
  Constant/1 -> Divide/2
  in/1 -> Sum/1
  Integrator/1 -> out/1, Sum/2  "A"
  Divide/1 -> Integrator/1  "dA"
  Sum/1 -> Divide/1

== system nms_sim_2D_cost/CPG-reflex-synergy controller/Reflexes2/IN RC45 ==
  in : Inport
  Constant : Constant  Value=tau_act_diRusso
  Divide : Product  Inputs=*/
  Integrator : Integrator  InitialCondition=init_exc
  Sum : Sum  Inputs=+-|
  out : Outport  VectorParamsAs1DForOutWhenUnconnected=off
  wires:
  Constant/1 -> Divide/2
  in/1 -> Sum/1
  Integrator/1 -> out/1, Sum/2  "A"
  Divide/1 -> Integrator/1  "dA"
  Sum/1 -> Divide/1

== system nms_sim_2D_cost/CPG-reflex-synergy controller/Reflexes2/IN RC46 ==
  in : Inport
  Constant : Constant  Value=tau_act_diRusso
  Divide : Product  Inputs=*/
  Integrator : Integrator  InitialCondition=init_exc
  Sum : Sum  Inputs=+-|
  out : Outport  VectorParamsAs1DForOutWhenUnconnected=off
  wires:
  Constant/1 -> Divide/2
  in/1 -> Sum/1
  Integrator/1 -> out/1, Sum/2  "A"
  Divide/1 -> Integrator/1  "dA"
  Sum/1 -> Divide/1

== system nms_sim_2D_cost/CPG-reflex-synergy controller/Reflexes2/IN RC47 ==
  in : Inport
  Constant : Constant  Value=tau_act_diRusso
  Divide : Product  Inputs=*/
  Integrator : Integrator  InitialCondition=init_exc
  Sum : Sum  Inputs=+-|
  out : Outport  VectorParamsAs1DForOutWhenUnconnected=off
  wires:
  Constant/1 -> Divide/2
  in/1 -> Sum/1
  Integrator/1 -> out/1, Sum/2  "A"
  Divide/1 -> Integrator/1  "dA"
  Sum/1 -> Divide/1

== system nms_sim_2D_cost/CPG-reflex-synergy controller/Reflexes2/IN RC48 ==
  in : Inport
  Constant : Constant  Value=tau_act_diRusso
  Divide : Product  Inputs=*/
  Integrator : Integrator  InitialCondition=init_exc
  Sum : Sum  Inputs=+-|
  out : Outport  VectorParamsAs1DForOutWhenUnconnected=off
  wires:
  Constant/1 -> Divide/2
  in/1 -> Sum/1
  Integrator/1 -> out/1, Sum/2  "A"
  Divide/1 -> Integrator/1  "dA"
  Sum/1 -> Divide/1

== system nms_sim_2D_cost/CPG-reflex-synergy controller/Reflexes2/IN RC49 ==
  in : Inport
  Constant : Constant  Value=tau_act_diRusso
  Divide : Product  Inputs=*/
  Integrator : Integrator  InitialCondition=init_exc
  Sum : Sum  Inputs=+-|
  out : Outport  VectorParamsAs1DForOutWhenUnconnected=off
  wires:
  Constant/1 -> Divide/2
  in/1 -> Sum/1
  Integrator/1 -> out/1, Sum/2  "A"
  Divide/1 -> Integrator/1  "dA"
  Sum/1 -> Divide/1

== system nms_sim_2D_cost/CPG-reflex-synergy controller/Reflexes2/IN RC5 ==
  in : Inport
  Constant : Constant  Value=tau_act_diRusso
  Divide : Product  Inputs=*/
  Integrator : Integrator  InitialCondition=init_exc
  Sum : Sum  Inputs=+-|
  out : Outport  VectorParamsAs1DForOutWhenUnconnected=off
  wires:
  Constant/1 -> Divide/2
  in/1 -> Sum/1
  Integrator/1 -> out/1, Sum/2  "A"
  Divide/1 -> Integrator/1  "dA"
  Sum/1 -> Divide/1

== system nms_sim_2D_cost/CPG-reflex-synergy controller/Reflexes2/IN RC50 ==
  in : Inport
  Constant : Constant  Value=tau_act_diRusso
  Divide : Product  Inputs=*/
  Integrator : Integrator  InitialCondition=init_exc
  Sum : Sum  Inputs=+-|
  out : Outport  VectorParamsAs1DForOutWhenUnconnected=off
  wires:
  Constant/1 -> Divide/2
  in/1 -> Sum/1
  Integrator/1 -> out/1, Sum/2  "A"
  Divide/1 -> Integrator/1  "dA"
  Sum/1 -> Divide/1

== system nms_sim_2D_cost/CPG-reflex-synergy controller/Reflexes2/IN RC51 ==
  in : Inport
  Constant : Constant  Value=tau_act_diRusso
  Divide : Product  Inputs=*/
  Integrator : Integrator  InitialCondition=init_exc
  Sum : Sum  Inputs=+-|
  out : Outport  VectorParamsAs1DForOutWhenUnconnected=off
  wires:
  Constant/1 -> Divide/2
  in/1 -> Sum/1
  Integrator/1 -> out/1, Sum/2  "A"
  Divide/1 -> Integrator/1  "dA"
  Sum/1 -> Divide/1

== system nms_sim_2D_cost/CPG-reflex-synergy controller/Reflexes2/IN RC6 ==
  in : Inport
  Constant : Constant  Value=tau_act_diRusso
  Divide : Product  Inputs=*/
  Integrator : Integrator  InitialCondition=init_exc
  Sum : Sum  Inputs=+-|
  out : Outport  VectorParamsAs1DForOutWhenUnconnected=off
  wires:
  Constant/1 -> Divide/2
  in/1 -> Sum/1
  Integrator/1 -> out/1, Sum/2  "A"
  Divide/1 -> Integrator/1  "dA"
  Sum/1 -> Divide/1

== system nms_sim_2D_cost/CPG-reflex-synergy controller/Reflexes2/IN RC7 ==
  in : Inport
  Constant : Constant  Value=tau_act_diRusso
  Divide : Product  Inputs=*/
  Integrator : Integrator  InitialCondition=init_exc
  Sum : Sum  Inputs=+-|
  out : Outport  VectorParamsAs1DForOutWhenUnconnected=off
  wires:
  Constant/1 -> Divide/2
  in/1 -> Sum/1
  Integrator/1 -> out/1, Sum/2  "A"
  Divide/1 -> Integrator/1  "dA"
  Sum/1 -> Divide/1

== system nms_sim_2D_cost/CPG-reflex-synergy controller/Reflexes2/IN RC8 ==
  in : Inport
  Constant : Constant  Value=tau_act_diRusso
  Divide : Product  Inputs=*/
  Integrator : Integrator  InitialCondition=init_exc
  Sum : Sum  Inputs=+-|
  out : Outport  VectorParamsAs1DForOutWhenUnconnected=off
  wires:
  Sum/1 -> Divide/1
  Divide/1 -> Integrator/1  "dA"
  Integrator/1 -> Sum/2, out/1  "A"
  in/1 -> Sum/1
  Constant/1 -> Divide/2

== system nms_sim_2D_cost/CPG-reflex-synergy controller/Reflexes2/IN RC9 ==
  in : Inport
  Constant : Constant  Value=tau_act_diRusso
  Divide : Product  Inputs=*/
  Integrator : Integrator  InitialCondition=init_exc
  Sum : Sum  Inputs=+-|
  out : Outport  VectorParamsAs1DForOutWhenUnconnected=off
  wires:
  Constant/1 -> Divide/2
  in/1 -> Sum/1
  Integrator/1 -> out/1, Sum/2  "A"
  Divide/1 -> Integrator/1  "dA"
  Sum/1 -> Divide/1

== system nms_sim_2D_cost/CPG-reflex-synergy controller/Reflexes2/SN ==
  In1 : Inport
  Gain : Gain  Gain=65/200
  Sqrt : Sqrt
  Out1 : Outport
  wires:
  In1/1 -> Sqrt/1
  Sqrt/1 -> Gain/1
  Gain/1 -> Out1/1

== system nms_sim_2D_cost/CPG-reflex-synergy controller/Reflexes2/SN1 ==
  In1 : Inport
  Gain : Gain  Gain=65/200
  Sqrt : Sqrt
  Out1 : Outport
  wires:
  Gain/1 -> Out1/1
  Sqrt/1 -> Gain/1
  In1/1 -> Sqrt/1

== system nms_sim_2D_cost/CPG-reflex-synergy controller/Reflexes2/SN2 ==
  In1 : Inport
  Gain : Gain  Gain=65/200
  Sqrt : Sqrt
  Out1 : Outport
  wires:
  In1/1 -> Sqrt/1
  Sqrt/1 -> Gain/1
  Gain/1 -> Out1/1

== system nms_sim_2D_cost/CPG-reflex-synergy controller/Reflexes2/SN3 ==
  In1 : Inport
  Gain : Gain  Gain=65/200
  Sqrt : Sqrt
  Out1 : Outport
  wires:
  Gain/1 -> Out1/1
  Sqrt/1 -> Gain/1
  In1/1 -> Sqrt/1

== system nms_sim_2D_cost/CPG-reflex-synergy controller/Reflexes2/SN4 ==
  In1 : Inport
  Gain : Gain  Gain=65/200
  Sqrt : Sqrt
  Out1 : Outport
  wires:
  In1/1 -> Sqrt/1
  Sqrt/1 -> Gain/1
  Gain/1 -> Out1/1

== system nms_sim_2D_cost/CPG-reflex-synergy controller/Reflexes2/SN5 ==
  In1 : Inport
  Gain : Gain  Gain=65/200
  Sqrt : Sqrt
  Out1 : Outport
  wires:
  Gain/1 -> Out1/1
  Sqrt/1 -> Gain/1
  In1/1 -> Sqrt/1

== system nms_sim_2D_cost/CPG-reflex-synergy controller/Reflexes2/SN6 ==
  In1 : Inport
  Gain : Gain  Gain=65/200
  Sqrt : Sqrt
  Out1 : Outport
  wires:
  In1/1 -> Sqrt/1
  Sqrt/1 -> Gain/1
  Gain/1 -> Out1/1

== system nms_sim_2D_cost/CPG-reflex-synergy controller/Reflexes2/SN7 ==
  In1 : Inport
  Gain : Gain  Gain=65/200
  Sqrt : Sqrt
  Out1 : Outport
  wires:
  Gain/1 -> Out1/1
  Sqrt/1 -> Gain/1
  In1/1 -> Sqrt/1

== system nms_sim_2D_cost/CPG-reflex-synergy controller/Reflexes2/SN8 ==
  In1 : Inport
  Gain : Gain  Gain=65/200
  Sqrt : Sqrt
  Out1 : Outport
  wires:
  In1/1 -> Sqrt/1
  Sqrt/1 -> Gain/1
  Gain/1 -> Out1/1
